simulink model "practica2_1_derivativo_proportional_integral"  (R2026b)
settings: Solver=VariableStepAuto  StopTime=60
settings Model: Creator=diego  LastModifiedBy=ivanp

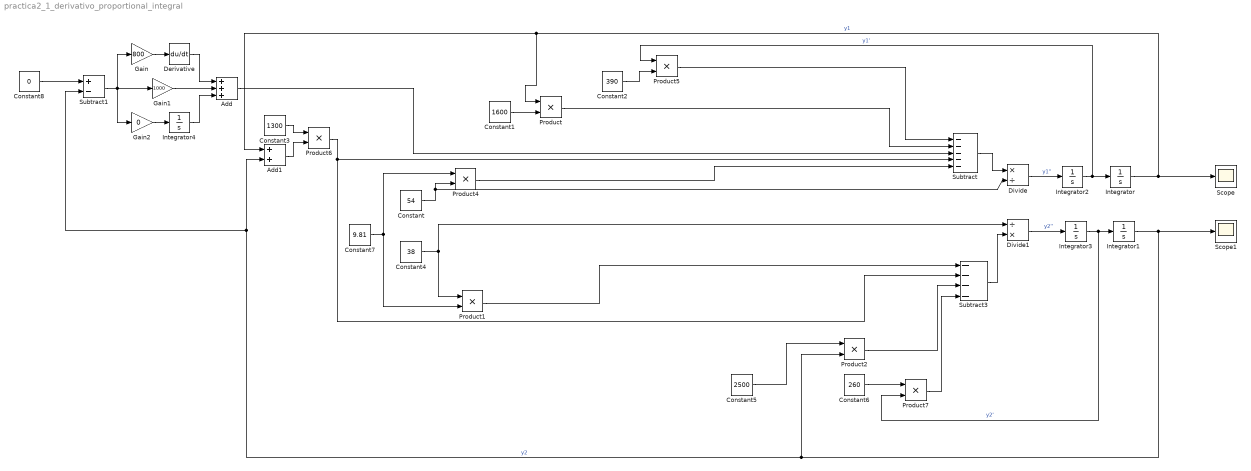
== system practica2_1_derivativo_proportional_integral ==
  Add : Sum  Inputs=+++
  Add1 : Sum
  Constant : Constant  Value=54
  Constant1 : Constant  Value=1600
  Constant2 : Constant  Value=390
  Constant3 : Constant  Value=1300
  Constant4 : Constant  Value=38
  Constant5 : Constant  Value=2500
  Constant6 : Constant  Value=260
  Constant7 : Constant  Value=9.81
  Constant8 : Constant  Value=0
  Derivative : Derivative
  Divide : Product  Inputs=*/
  Divide1 : Product  Inputs=/*
  Gain : Gain  Gain=800
  Gain1 : Gain  Gain=1000
  Gain2 : Gain  Gain=0
  Integrator{,1..4} (5 alike) : Integrator
  Product{,1..2,4..7} (7 alike) : Product
  Scope : Scope
      settings: ActiveDisplayYMinimum=-0.17918114939757934  ActiveDisplayYMaximum=-0.1784720639573012
  Scope1 : Scope
      settings: ActiveDisplayYMinimum=-0.037147167372447859  ActiveDisplayYMaximum=-0.036718178948774841
  Subtract : Sum  Inputs=-----
  Subtract1 : Sum  Inputs=+-
  Subtract3 : Sum  Inputs=----
  wires:
  Integrator/1 -> Add1/1, Product/1, Scope/1  "y1"
  Integrator1/1 -> Product2/2, Subtract1/2, Add1/2, Scope1/1  "y2"
  Integrator2/1 -> Product5/1, Integrator/1  "y1'"
  Integrator3/1 -> Product7/2, Integrator1/1  "y2'"
  Divide/1 -> Integrator2/1  "y1''"
  Divide1/1 -> Integrator3/1  "y2''"
  Constant/1 -> Product4/2, Divide/2
  Constant4/1 -> Product1/1, Divide1/1
  Subtract/1 -> Divide/1
  Subtract3/1 -> Divide1/2
  Constant1/1 -> Product/2
  Product5/1 -> Subtract/1
  Constant7/1 -> Product1/2, Product4/1
  Product1/1 -> Subtract3/1
  Constant3/1 -> Product6/1
  Add1/1 -> Product6/2
  Product6/1 -> Subtract/4, Subtract3/2
  Product7/1 -> Subtract3/4
  Product2/1 -> Subtract3/3
  Constant5/1 -> Product2/1
  Constant6/1 -> Product7/1
  Product4/1 -> Subtract/5
  Constant2/1 -> Product5/2
  Product/1 -> Subtract/2
  Constant8/1 -> Subtract1/1
  Subtract1/1 -> Gain1/1, Gain/1, Gain2/1
  Derivative/1 -> Add/1
  Gain/1 -> Derivative/1
  Add/1 -> Subtract/3
  Gain1/1 -> Add/2
  Gain2/1 -> Integrator4/1
  Integrator4/1 -> Add/3
